simulink model "AULA2"  (R2025b)
settings: Solver=VariableStepAuto  StartTime=0.0  StopTime=100  RelTol=1e-3
settings Model: Creator=RA00338338  LastModifiedBy=RA00338338

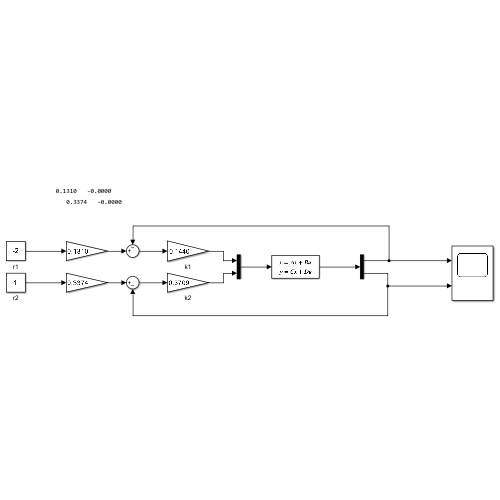
[thumbnail: Simulink's stored preview of the top-level diagram]
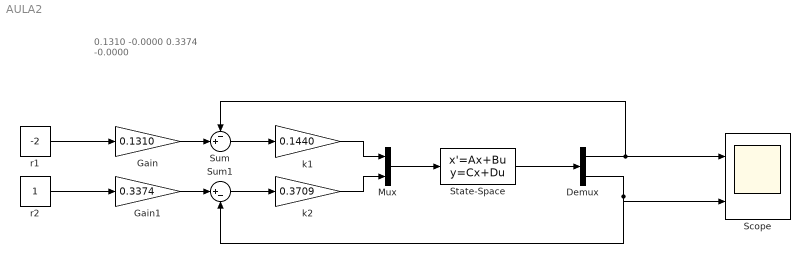
== system AULA2 ==
  note: 0.1310 -0.0000
      | 0.3374 -0.0000
  Demux : Demux  Outputs=2
  Gain : Gain  Gain=0.1310
  Gain1 : Gain  Gain=0.3374
  Mux : Mux  Inputs=2
  Scope : Scope  NumInputPorts=2
      settings: ActiveDisplayYMinimum=-0.11271166530636857  ActiveDisplayYMaximum=0.79682582501088761
  State-Space : StateSpace  A="[ 0  1; 0  0 ]"  B="[ 0  0; 1  1 ]"  C=eye(2,2)  D=zeros(2,2)  InitialCondition=0
  Sum : Sum  Inputs=-+|
  Sum1 : Sum  Inputs=|+-
  k1 : Gain  Gain=0.1440
  k2 : Gain  Gain=0.3709
  r1 : Constant  Value=-2
  r2 : Constant
  wires:
  Mux/1 -> State-Space/1
  k2/1 -> Mux/2
  k1/1 -> Mux/1
  Sum/1 -> k1/1
  Sum1/1 -> k2/1
  State-Space/1 -> Demux/1
  Demux/1 -> Sum/1, Scope/1
  Demux/2 -> Sum1/2, Scope/2
  r1/1 -> Gain/1
  r2/1 -> Gain1/1
  Gain/1 -> Sum/2
  Gain1/1 -> Sum1/1
